simulink model "pendulum_RL"  (R2026a)
settings: Solver=VariableStepAuto  StopTime=15
values from neighbouring files (symbols this model uses):
  p = [ ... (first row only)    [init_pendulum.m]
  q0 = [ ... (first row only)    [init_pendulum.m]
  qd0 = [ ... (first row only)    [init_pendulum.m]
  trainingMode = 0    [init_pendulum.m]    (also in rl_v3_cont.m; rl_v4_cont.m; train_RL_V4.m)
  Ts = 0.02    [RL_SAC_V2_wv3_300ep.mat]    (also in setup_RL.m; train_RL_V2.m; train_RL_V4.m)
  vTrainCmd = 0    [init_pendulum.m]
libraries: rllib x1
settings Model: Creator=vb  LastModifiedBy=User

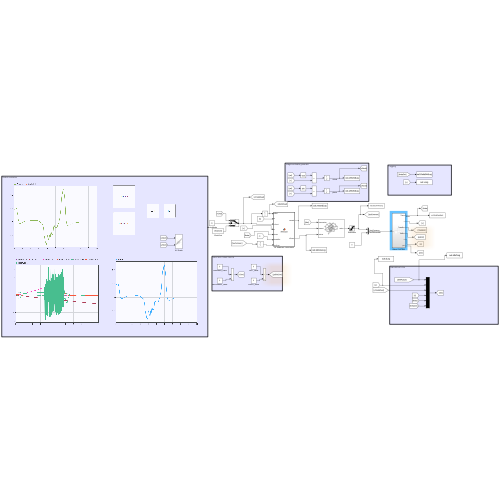
[thumbnail: Simulink's stored preview of the top-level diagram]
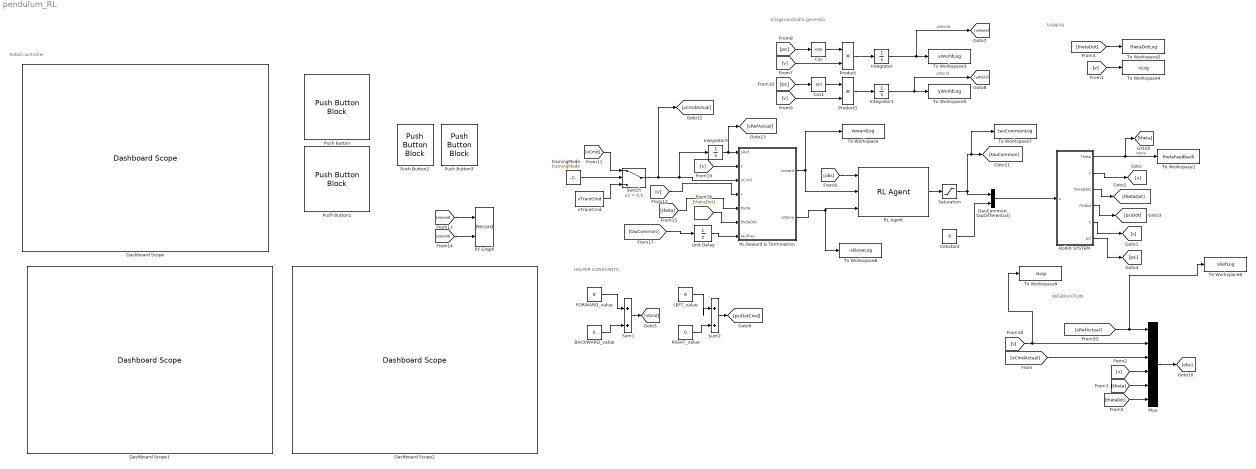
== system pendulum_RL ==
  note: OBSERVATION
  note: HELPER CONSTANTS
  note: Robot controller
  note: Világkoordináta generáló
  note: Logging
  BACKWARD_value : Constant  Value=0
  Constant : Constant  Value=0
  Cos : Trigonometry  Operator=cos
  Cos1 : Trigonometry
  Dashboard Scope : DashboardScope  FontColor=[0.0, 0.0, 0.0]
  Dashboard Scope1 : DashboardScope  FontColor=[0.0, 0.0, 0.0]
  Dashboard Scope2 : DashboardScope  FontColor=[0.0, 0.0, 0.0]
  FORWARD_value : Constant  Value=0
  Integrator : Integrator
  Integrator1 : Integrator
  Integrator3 : Integrator
  LEFT_value : Constant  Value=0
  Mux : Mux  Inputs=6
  Product : Product
  Product1 : Product
  Push Button : PushButtonBlock  ButtonText=FORWARD  OnValue=0.15  IconOnColor=[0.0, 0.39215686274509803, 0.0]  IconOffColor=[0.0, 1.0, 0.0]  OffValue=0.000000
  Push Button1 : PushButtonBlock  ButtonText=BACKWARD  OnValue=-0.15  IconOnColor=[0.0, 0.39215686274509803, 0.0]  IconOffColor=[0.0, 1.0, 0.0]  OffValue=0.000000
  Push Button2 : PushButtonBlock  ButtonText=LEFT  OnValue=+0.5236  IconOnColor=[0.0, 0.39215686274509803, 0.0]  IconOffColor=[0.0, 1.0, 0.0]  OffValue=0.000000
  Push Button3 : PushButtonBlock  ButtonText=RIGHT  OnValue=-0.5236  IconOnColor=[0.0, 0.39215686274509803, 0.0]  IconOffColor=[0.0, 1.0, 0.0]  OffValue=0.000000
  RIGHT_value : Constant  Value=0
  RL Agent : rllib/RL Agent  Agent=agent  ExternalActionAsInput=off  ProvideLastAction=off  ProvideCumRwd=off  TreatAsDirectFeedthrough=on  UseStrictObservationDataTypes=off
  RL Reward & Termination : MATLAB Function  TreatAsAtomicUnit=on
  Robot SYSTEM : Subsystem
  Saturation : Saturate  UpperLimit=2  LowerLimit=-2
  Sum1 : Sum  Inputs=|++
  Sum2 : Sum  Inputs=|++
  Switch : Switch  Criteria=u2 > Threshold  Threshold=0.5  SaturateOnIntegerOverflow=off  InputSameDT=off
  To Workspace : ToWorkspace  VariableName=rewardLog  SaveFormat=Timeseries  SampleTime=-1
  To Workspace1 : ToWorkspace  VariableName=thetaFeedback  SaveFormat=Timeseries  SampleTime=-1
  To Workspace2 : ToWorkspace  VariableName=thetaDotLog  SaveFormat=Timeseries  SampleTime=-1
  To Workspace3 : ToWorkspace  VariableName=xWorldLog  SaveFormat=Timeseries  SampleTime=-1
  To Workspace4 : ToWorkspace  VariableName=vLog  SaveFormat=Timeseries  SampleTime=-1
  To Workspace5 : ToWorkspace  VariableName=yWorldLog  SaveFormat=Timeseries  SampleTime=-1
  To Workspace6 : ToWorkspace  VariableName=isDoneLog  SaveFormat=Timeseries  SampleTime=-1
  To Workspace7 : ToWorkspace  VariableName=tauCommonLog  SaveFormat=Timeseries  SampleTime=-1
  To Workspace8 : ToWorkspace  VariableName=sRefLog  SaveFormat=Timeseries  SampleTime=-1
  To Workspace9 : ToWorkspace  VariableName=sLog  SaveFormat=Timeseries  SampleTime=-1
  Unit Delay : UnitDelay  SampleTime=Ts
  XY Graph : Record  NumPorts=2.0  FileSettingsInternal="{\"entries\":[{\"content\":{\"excelSettings\":{\"content\":{},\"type\":\"Streamout.ExcelSettings\"},\"parquetSettings\":{\"content\":{},\"type\":\"Streamout.ParquetSettings\"}},\"type\":\"Streamout.FileSettingStorage\",\"uuid\":\"\"}],\"packageUris\":[\"http:\\/\\/schema.mathworks.com\\/mf0\\/streamout_blocks\\/R2020a\"],\"version\":\"1.0\"}"  FrameSettings=[0, 0]  Layout=[1 1]  SignalsInternal="{\"entries\":[{\"content\":{\"signals\":[{\"content\":{\"blockPath\":[],\"dimensions\":[1,1],\"domain\":\"\",\"lineColor\":\"#a2142f\",\"plots\":[ 1 ],\"port\":1,\"sid\":[\"\"],\"signalID\":1,\"signalName\":\"From13\"},\"type\":\"RecordBlkView.Signal\",\"uuid\":\"\"},{\"content\":{\"blockPath\":[],\"dimensions\":[1,1],\"domain\":\"\",\"lineColor\":\"#139fff\",\"plots\":[ 1 ],\"port\":2,\"sid\":[\"\"],\"signalID\":2,\"signalName\":\"From14\"},\"type\":\"RecordBlkView.Signal\",\"uuid\":\"\"}]},\"type\":\"RecordBlkView.InputSignals\",\"uuid\":\"\"}],\"packageUris\":[\"http:\\/\\/schema.mathworks.com\\/mf0\\/streamout_blocks\\/R2020a\"],\"version\":\"1.0\"}"  VisualizationBindings="{\"xyplotplugin\":{\"info\":[{\"series\":[{\"bindingParametersList\":[{\"parameter\":\"X-Axis\",\"signalID\":1,\"signalName\":\"From13\"},{\"parameter\":\"Y-Axis\",\"signalID\":2,\"signalName\":\"From14\"}],\"seriesID\":0}],\"subplotID\":1}]}}"  CompatibilityTag=XY
  "[tauCommon, tauDifferential]" : Mux  Inputs=2
  trainingMode : Constant  Value=trainingMode
  vTrainCmd : Constant  Value=vTrainCmd
  wires:
  Robot SYSTEM/1(Theta) -> [theta], To Workspace1/1  "theta"
  "[tauCommon, tauDifferential]"/1 -> Robot SYSTEM/1(u)
  Robot SYSTEM/2(v) -> [v]
  [v] -> To Workspace4/1
  Robot SYSTEM/5(s) -> [s]
  Robot SYSTEM/3(ThetaDot) -> [thetaDot]
  [thetaDot] -> To Workspace2/1
  Robot SYSTEM/4(PsiDot) -> [psiDot]
  Robot SYSTEM/6(psi) -> [psi]
  Cos/1 -> Product/1
  [v] -> Product/2
  [psi] -> Cos/1
  Product/1 -> Integrator/1
  Integrator/1 -> [xWorld], To Workspace3/1  "xWorld"
  Integrator1/1 -> [yWorld], To Workspace5/1  "yWorld"
  Cos1/1 -> Product1/1
  [psi] -> Cos1/1
  Product1/1 -> Integrator1/1
  [v] -> Product1/2
  FORWARD_value/1 -> Sum1/1
  BACKWARD_value/1 -> Sum1/2
  Sum1/1 -> [vCmd]
  Sum2/1 -> [psiDotCmd]
  LEFT_value/1 -> Sum2/1
  RIGHT_value/1 -> Sum2/2
  [xWorld] -> XY Graph/1
  [yWorld] -> XY Graph/2
  Constant/1 -> "[tauCommon, tauDifferential]"/2
  Mux/1 -> [obs]
  [obs] -> RL Agent/1
  RL Agent/1 -> Saturation/1
  Saturation/1 -> "[tauCommon, tauDifferential]"/1, To Workspace7/1, [tauCommon]
  RL Reward & Termination/1(reward) -> To Workspace/1, RL Agent/2
  RL Reward & Termination/2(isDone) -> To Workspace6/1, RL Agent/3
  [v] -> RL Reward & Termination/4(v)
  [theta] -> RL Reward & Termination/5(theta)
  [thetaDot] -> RL Reward & Termination/6(thetaDot)
  Switch/1 -> [vCmdActual], Integrator3/1, RL Reward & Termination/3(vCmd)
  [vCmd] -> Switch/1
  vTrainCmd/1 -> Switch/3
  trainingMode/1 -> Switch/2
  Unit Delay/1 -> RL Reward & Termination/7(tauPrev)
  [tauCommon] -> Unit Delay/1
  [v] -> Mux/4
  [vCmdActual] -> Mux/3
  [theta] -> Mux/5
  [thetaDot] -> Mux/6
  [s] -> To Workspace9/1, Mux/2
  [s] -> RL Reward & Termination/2(s)
  Integrator3/1 -> [sRefActual], RL Reward & Termination/1(sRef)
  [sRefActual] -> Mux/1, To Workspace8/1

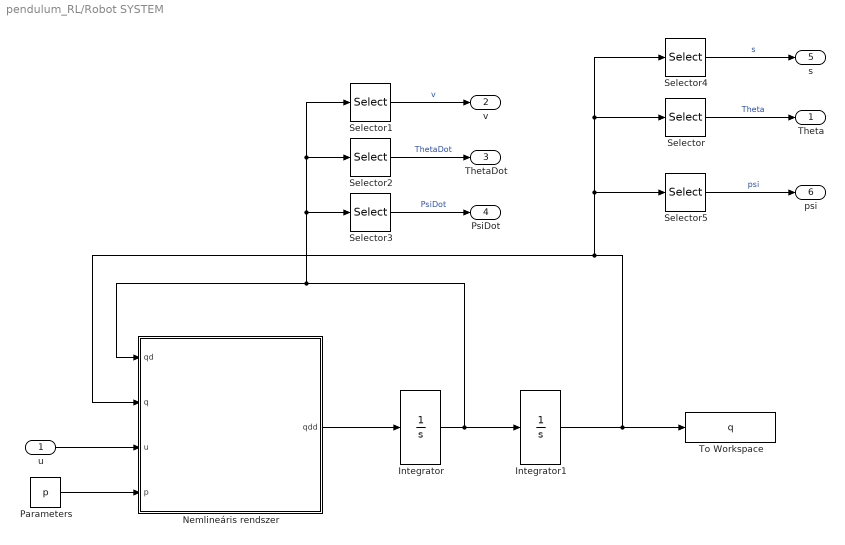
== system pendulum_RL/Robot SYSTEM ==
  u : Inport
  Integrator : Integrator  InitialCondition=qd0
  Integrator1 : Integrator  InitialCondition=q0
  Nemlineáris rendszer : MATLAB Function  TreatAsAtomicUnit=on
  Parameters : Constant  Value=p
  Selector : Selector  InputPortWidth=3  IndexOptions=Index vector (dialog)  Indices=2  OutputSizes=1
  Selector1 : Selector  InputPortWidth=3  IndexOptions=Index vector (dialog)  Indices=1  OutputSizes=1
  Selector2 : Selector  InputPortWidth=3  IndexOptions=Index vector (dialog)  Indices=2  OutputSizes=1
  Selector3 : Selector  InputPortWidth=3  IndexOptions=Index vector (dialog)  Indices=3  OutputSizes=1
  Selector4 : Selector  InputPortWidth=3  IndexOptions=Index vector (dialog)  Indices=1  OutputSizes=1
  Selector5 : Selector  InputPortWidth=3  IndexOptions=Index vector (dialog)  Indices=3  OutputSizes=1
  To Workspace : ToWorkspace  VariableName=q  SaveFormat=Timeseries  SampleTime=-1
  Theta : Outport
  v : Outport  Port=2
  ThetaDot : Outport  Port=3
  PsiDot : Outport  Port=4
  s : Outport  Port=5
  psi : Outport  Port=6
  wires:
  Selector/1 -> Theta/1  "Theta"
  Integrator1/1 -> To Workspace/1, Selector5/1, Selector/1, Selector4/1, Nemlineáris rendszer/2(q)
  Selector1/1 -> v/1  "v"
  Nemlineáris rendszer/1(qdd) -> Integrator/1
  u/1 -> Nemlineáris rendszer/3(u)
  Selector2/1 -> ThetaDot/1  "ThetaDot"
  Selector3/1 -> PsiDot/1  "PsiDot"
  Parameters/1 -> Nemlineáris rendszer/4(p)
  Integrator/1 -> Selector2/1, Selector1/1, Selector3/1, Nemlineáris rendszer/1(qd), Integrator1/1
  Selector4/1 -> s/1  "s"
  Selector5/1 -> psi/1  "psi"

== matlab function pendulum_RL/RL Reward & Termination ==
  data: sRef input; s input; vCmd input; reward output; v input; theta input; thetaDot input; tauPrev input; isDone output
function [reward, isDone] = rlReward( ...
    sRef, s, vCmd, v, theta, thetaDot, tauPrev)

    %% Normalizálási skálák
    sScale        = 0.5;           % [m]
    vScale        = 0.2;           % [m/s]
    thetaScale    = 10*pi/180;     % [rad]
    thetaDotScale = 2.0;           % [rad/s]
    tauScale      = 2.0;           % [Nm]

    %% Normalizált hibák / állapotok
    eS        = (sRef - s) / sScale;
    eV        = (vCmd - v) / vScale;
    thetaN    = theta / thetaScale;
    thetaDotN = thetaDot / thetaDotScale;
    tauN      = tauPrev / tauScale;

    %% Cost
    cost = ...
          1  * eS^2 ...
        + 1.0  * eV^2 ...
        + 4.0  * thetaN^2 ...
        + 0.25 * thetaDotN^2 ...
        + 0.02 * tauN^2;

    %% Reward
    reward = 1.0 - cost;

    %% Elesés
    fallAngle = 30*pi/180;

    isDone = abs(theta) > fallAngle;

    if isDone
        reward = -100;
    end
end

== matlab function pendulum_RL/Robot SYSTEM/Nemlineáris rendszer ==
  data: qd input; q input; u input; qdd output; p input
function qdd = nonlinearDynamics(qd, q, u, p)

% q  = [s, theta, psi]
% qd = [v, thetaDot, psiDot]
% u  = [tauCommon, tauDifferential]

%% Alap fizikai paraméterek

mb  = p(1);
mw  = p(2);
r   = p(3);
b   = p(4);
l   = p(5);

Ix  = p(6);
Iy  = p(7);
Iz  = p(8);

Ja  = p(9);
Jzw = p(10);

g   = p(11);

%% Súrlódási / veszteségi paraméterek

cMotor   = p(12);   % motor+csapágy viszkózus súrlódás [Nms/rad]
tauMotor = p(13);   % motor+csapágy Coulomb súrlódás [Nm]

cRoll    = p(14);   % gördülési viszkózus ellenállás [Ns/m]
FRoll    = p(15);   % gördülési Coulomb jellegű ellenállás [N]

cAir     = p(16);   % légellenállási együttható

vEps     = p(17);   % simítási sebesség [m/s]
omegaEps = p(18);   % simítási szögsebesség [rad/s]


%% Állapotok

v        = qd(1);
theta    = q(2);
thetaDot = qd(2);
psiDot   = qd(3);


%% Összevont tehetetlenségek

A = mb + 2*mw + 2*Ja/r^2;

C = Iy + mb*l^2;

D = Ix*sin(theta)^2 ...
  + Iz*cos(theta)^2 ...
  + mb*l^2*sin(theta)^2 ...
  + mw*b^2/2 ...
  + Ja*b^2/(2*r^2) ...
  + 2*Jzw;

Dp = 2*sin(theta)*cos(theta) ...
   * (Ix - Iz + mb*l^2);


%% Tömegmátrix

M = [
    A,                  mb*l*cos(theta), 0;
    mb*l*cos(theta),    C,               0;
    0,                  0,               D
];


%% Nemlineáris konzervatív tagok

h = [
    -mb*l*sin(theta)*thetaDot^2;
    -0.5*Dp*psiDot^2 - mb*g*l*sin(theta);
    Dp*thetaDot*psiDot
];


%% Bemeneti mátrix

B = [
     2/r, 0;
    -2,   0;
     0,   b/r
];


%% ------------------------------------------------------------
% Keréksebességek
% ------------------------------------------------------------

vL = v - b/2*psiDot;
vR = v + b/2*psiDot;

omegaL = vL/r;
omegaR = vR/r;


%% ------------------------------------------------------------
% Motor / csapágy relatív szögsebességek
% ------------------------------------------------------------

alphaDotL = omegaL - thetaDot;
alphaDotR = omegaR - thetaDot;


%% ------------------------------------------------------------
% Motor + csapágy súrlódási nyomaték
% ------------------------------------------------------------

tauFricL = cMotor*alphaDotL ...
         + tauMotor*tanh(alphaDotL/omegaEps);

tauFricR = cMotor*alphaDotR ...
         + tauMotor*tanh(alphaDotR/omegaEps);


% közös / különbségi komponensek

tauFricCommon = (tauFricL + tauFricR)/2;
tauFricDiff   = (tauFricR - tauFricL)/2;

uFric = [
    tauFricCommon;
    tauFricDiff
];

QmotorFric = -B*uFric;


%% ------------------------------------------------------------
% Gördülési ellenállás
% ------------------------------------------------------------

FrollL = cRoll*vL ...
       + FRoll*tanh(vL/vEps);

FrollR = cRoll*vR ...
       + FRoll*tanh(vR/vEps);

Qroll = [
    -(FrollL + FrollR);
     0;
    -b/2*(FrollR - FrollL)
];


%% ------------------------------------------------------------
% Légellenállás
% ------------------------------------------------------------

Fair = cAir*v*abs(v);

Qair = [
    -Fair;
     0;
     0
];


%% ------------------------------------------------------------
% Teljes disszipatív általánosított erő
% ------------------------------------------------------------

Qfriction = QmotorFric + Qroll + Qair;


%% ------------------------------------------------------------
% Mozgásegyenlet
% ------------------------------------------------------------

qdd = M \ (B*u + Qfriction - h);

end
